simulink model "Exp10"  (R2025b)
settings: Solver=VariableStepAuto  StartTime=0.0  StopTime=10.0  RelTol=1e-3
libraries: hdlsllib x1
settings Model: Creator=SUBHASH  LastModifiedBy=SUBHASH

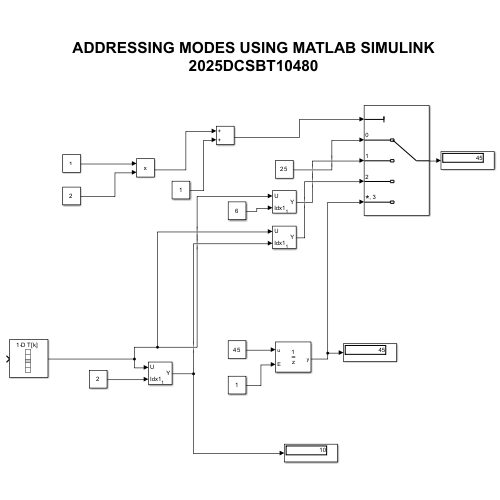
[thumbnail: Simulink's stored preview of the top-level diagram]
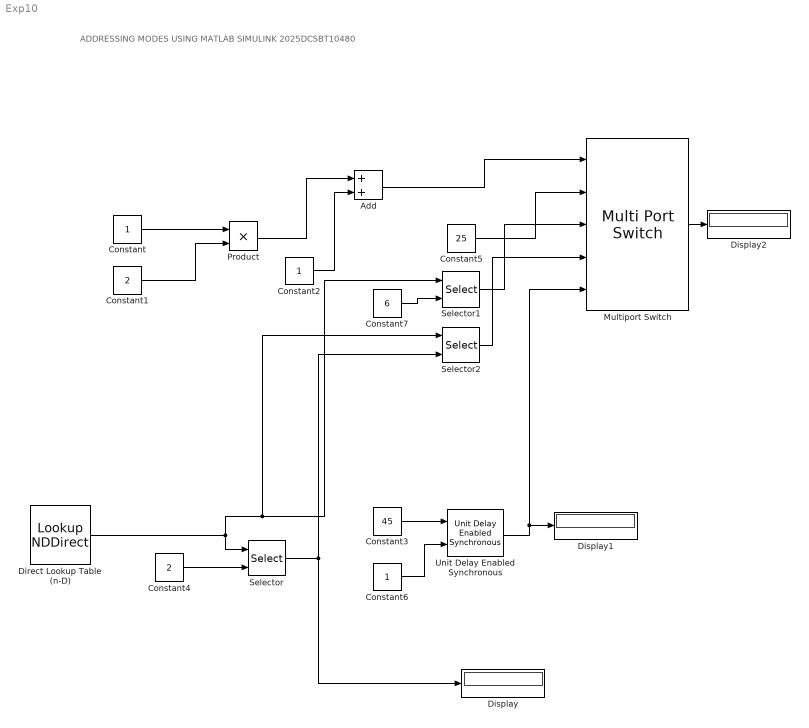
== system Exp10 ==
  note: ADDRESSING MODES USING MATLAB SIMULINK
      | 2025DCSBT10480
  Add : Sum
  Constant : Constant
  Constant1 : Constant  Value=2
  Constant2 : Constant
  Constant3 : Constant  Value=45
  Constant4 : Constant  Value=2
  Constant5 : Constant  Value=25
  Constant6 : Constant
  Constant7 : Constant  Value=6
  Direct Lookup Table (n-D) : LookupNDDirect  NumberOfTableDimensions=1  Table=[10 8 20 30 40 50 60 70 90 100]
  Display : Display
  Display1 : Display
  Display2 : Display
  Multiport Switch : MultiPortSwitch  DataPortOrder=Zero-based contiguous  Inputs=4  zeroidx=on  SaturateOnIntegerOverflow=off  InputSameDT=off
  Product : Product
  Selector : Selector  InputPortWidth=10  IndexOptions=Index vector (port)  Indices=[1 3]  OutputSizes=1
  Selector1 : Selector  InputPortWidth=10  IndexOptions=Index vector (port)  Indices=[1 3]  OutputSizes=1
  Selector2 : Selector  InputPortWidth=10  IndexOptions=Index vector (port)  Indices=[1 3]  OutputSizes=1
  Unit Delay Enabled Synchronous : hdlsllib/Discrete/Unit Delay Enabled Synchronous  InitialCondition=0.0  SampleTime=-1
  wires:
  Constant/1 -> Product/1
  Constant1/1 -> Product/2
  Product/1 -> Add/1
  Constant2/1 -> Add/2
  Add/1 -> Multiport Switch/1
  Constant5/1 -> Multiport Switch/2
  Multiport Switch/1 -> Display2/1
  Constant3/1 -> Unit Delay Enabled Synchronous/1
  Constant6/1 -> Unit Delay Enabled Synchronous/2
  Unit Delay Enabled Synchronous/1 -> Multiport Switch/5, Display1/1
  Selector1/1 -> Multiport Switch/3
  Selector2/1 -> Multiport Switch/4
  Constant4/1 -> Selector/2
  Direct Lookup Table (n-D)/1 -> Selector1/1, Selector2/1, Selector/1
  Constant7/1 -> Selector1/2
  Selector/1 -> Selector2/2, Display/1
